simulink model "ThrottleAMF"  (R2026a)
settings: Solver=VariableStepAuto
undefined symbols (not defined in the file): R
settings Model: Creator=flori  LastModifiedBy=flori

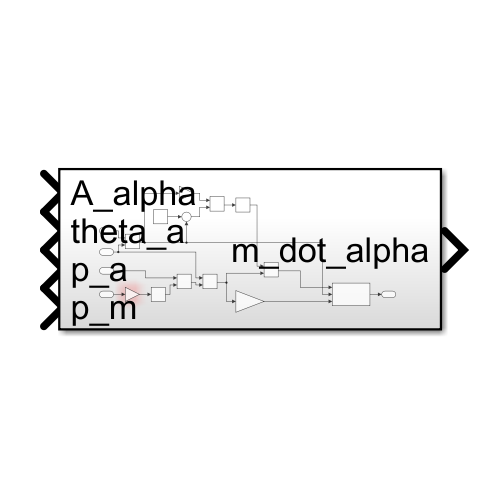
[thumbnail: Simulink's stored preview of the top-level diagram]
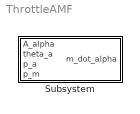
== system ThrottleAMF ==
  Subsystem : Subsystem

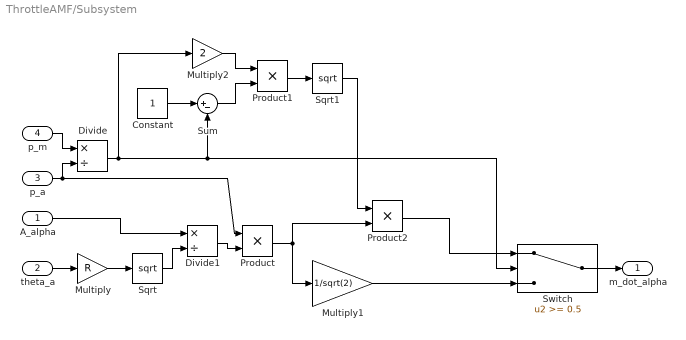
== system ThrottleAMF/Subsystem ==
  A_alpha : Inport
  theta_a : Inport  Port=2
  p_a : Inport  Port=3
  p_m : Inport  Port=4
  Constant : Constant
  Divide : Product  Inputs=*/
  Divide1 : Product  Inputs=*/
  Multiply : Gain  Gain=R
  Multiply1 : Gain  Gain=1/sqrt(2)
  Multiply2 : Gain  Gain=2
  Product : Product
  Product1 : Product
  Product2 : Product
  Sqrt : Sqrt
  Sqrt1 : Sqrt
  Sum : Sum  Inputs=|+-
  Switch : Switch  Threshold=0.5  SaturateOnIntegerOverflow=off  InputSameDT=off
  m_dot_alpha : Outport
  wires:
  Multiply/1 -> Sqrt/1
  Multiply2/1 -> Product1/1
  Divide/1 -> Switch/2, Sum/2, Multiply2/1
  A_alpha/1 -> Divide1/1
  p_m/1 -> Divide/1
  Sum/1 -> Product1/2
  Divide1/1 -> Product/2
  Product/1 -> Product2/2, Multiply1/1
  Constant/1 -> Sum/1
  Switch/1 -> m_dot_alpha/1
  theta_a/1 -> Multiply/1
  Multiply1/1 -> Switch/3
  Sqrt1/1 -> Product2/1
  Sqrt/1 -> Divide1/2
  Product1/1 -> Sqrt1/1
  p_a/1 -> Product/1, Divide/2
  Product2/1 -> Switch/1
